simulink model "series_hev_sf"  (R2026b)
settings: Solver=ode3  StopTime=tEnd  FixedStep=0.1
undefined symbols (not defined in the file): Qbat, SOC0, SOChigh, SOClow
settings Model: Creator=Hamza  LastModifiedBy=Hamza

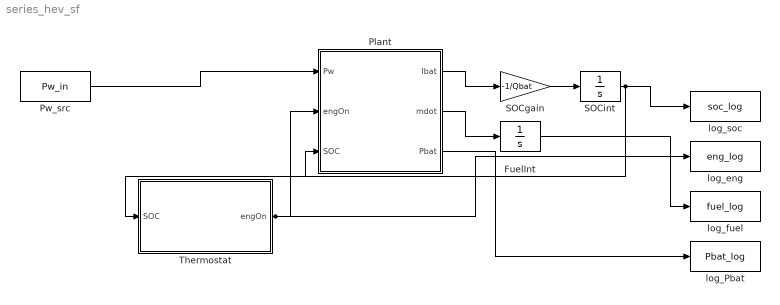
== system series_hev_sf ==
  FuelInt : Integrator
  Plant : MATLAB Function  TreatAsAtomicUnit=on
  Pw_src : FromWorkspace  VariableName=Pw_in
  SOCgain : Gain  Gain=-1/Qbat
  SOCint : Integrator  InitialCondition=SOC0
  Thermostat : Stateflow chart  TreatAsAtomicUnit=on
  log_Pbat : ToWorkspace  VariableName=Pbat_log  SaveFormat=Timeseries  SampleTime=-1
  log_eng : ToWorkspace  VariableName=eng_log  SaveFormat=Timeseries  SampleTime=-1
  log_fuel : ToWorkspace  VariableName=fuel_log  SaveFormat=Timeseries  SampleTime=-1
  log_soc : ToWorkspace  VariableName=soc_log  SaveFormat=Timeseries  SampleTime=-1
  wires:
  Pw_src/1 -> Plant/1(Pw)
  Thermostat/1(engOn) -> Plant/2(engOn), log_eng/1
  SOCint/1 -> Plant/3(SOC), Thermostat/1(SOC), log_soc/1
  Plant/1(Ibat) -> SOCgain/1
  SOCgain/1 -> SOCint/1
  Plant/2(mdot) -> FuelInt/1
  Plant/3(Pbat) -> log_Pbat/1
  FuelInt/1 -> log_fuel/1

== matlab function series_hev_sf/Plant ==
  data: Pw input; Ibat output; engOn input; SOC input; mdot output; Pbat output
function [Ibat, mdot, Pbat] = plant(Pw, engOn, SOC)
eta_m = 0.92; eta_g = 0.92; Paux = 500;
Pregen = 20e3; Pchg = 15e3; Pe_on = 20e3; Pe_max = 70e3;
LHV = 42.5e6; Rint = 0.15;
socTab = [0 0.2 0.4 0.6 0.8 1];
vocTab = [170 185 195 202 210 220];
loadFrac = [0 0.05 0.10 0.20 0.40 0.60 0.80 1.00];
eta_eng  = [0.05 0.14 0.20 0.27 0.33 0.34 0.33 0.31];
if Pw >= 0
    Pmot = Pw/eta_m;
else
    Pmot = max(Pw*eta_m, -Pregen);
end
Pbus = Pmot + Paux;
Peng = 0;
if engOn > 0.5, Peng = Pe_on; end
Pb = Pbus - Peng*eta_g;
Pb = max(Pb, -Pchg);
Voc = interp1(socTab, vocTab, min(max(SOC,0),1));
Pb = min(Pb, 0.99*Voc^2/(4*Rint));
Ibat = (Voc - sqrt(Voc^2 - 4*Rint*Pb))/(2*Rint);
Pbat = Pb;
mdot = 0;
if Peng > 0
    eta = interp1(loadFrac, eta_eng, Peng/Pe_max);
    mdot = Peng/(eta*LHV);
end
end

== stateflow chart series_hev_sf/Thermostat ==
  settings: updateMethod=DISCRETE  sampleTime=0.1
  state Engine_OFF
    entry: engOn = 0;
  state Engine_ON
    entry: engOn = 1;
  Engine_ON -> Engine_OFF : [SOC > SOChigh]
  (default) -> Engine_OFF
  Engine_OFF -> Engine_ON : [SOC < SOClow]
  data: SOC input; engOn output; SOClow parameter; SOChigh parameter
